simulink model "W07_wpt_los"  (R2024b)
settings: Solver=ode4  StartTime=0  StopTime=T_wpt  FixedStep=h  RelTol=1e-3
InitFcn:
  | addpath(fullfile(fileparts(fileparts(fileparts(get_param(bdroot, 'FileName')))), '_tools'), fileparts(get_param(bdroot, 'FileName'))); run_alone('W07', bdroot);
StopFcn:
  | W07_plot_wpt;
values from neighbouring files (symbols this model uses):
  alpha_lim = cfg.alpha_max(1)    [W07_0_setup.m]
  animate = 1    [W07_0_setup.m]    (also in W07_alloc_run.m = 0; W07_pose_run.m = 0; W07_wpt_run.m = 0)
  B_alloc = cfg.B    [W07_0_setup.m]
  beta_c = pi/2    (= 1.57079632679)    [W07_0_setup.m]
  Delta = 5    [W07_0_setup.m]
  eps_reg = 1e-4    (= 0.0001)    [W07_0_setup.m]    (also in W07_alloc_run.m)
  h = 0.02    [W07_0_setup.m]    (also in W07_3_build_wpt.m = add_line(sys, [a; via; b]); W07_4_build_pose.m = add_line(sys, [a; via; b]))
  k_neg = cfg.k_neg    [W07_0_setup.m]
  k_pos = cfg.k_pos    [W07_0_setup.m]
  Kb = 1    [W07_0_setup.m]
  Kd = 100    [W07_0_setup.m]
  Ki_u = 200    [W07_0_setup.m]
  Kp = 300    [W07_0_setup.m]
  Kp_u = 200    [W07_0_setup.m]
  mp = 25    [W07_0_setup.m]
  N_lim = 150    [W07_0_setup.m]
  n_max = cfg.n_max    [W07_0_setup.m]    (also in W07_plot_ca.m = base_num('n_max',      103.93); W07_plot_sat.m = base_var('n_max',      103.931))
  n_min = cfg.n_min    [W07_0_setup.m]    (also in W07_plot_ca.m = base_num('n_min',     -101.74); W07_plot_sat.m = base_var('n_min',     -101.737))
  Q_tau = eye(3)    [W07_0_setup.m]    (also in W07_alloc_run.m)
  quad = [cfg.pos ; cfg.alpha_max ; cfg.mount]    [W07_0_setup.m]
  R_switch = 3    [W07_0_setup.m]
  rp = [0.05 0 -0.35]'    [W07_0_setup.m]
  stop_at_end = 1    [W07_0_setup.m]
  stop_hold = 15    [W07_0_setup.m]
  T_neg = cfg.k_neg * cfg.n_min^2    [W07_0_setup.m]    (also in W07_plot_ca.m = base_num('T_neg',       66.708); W07_plot_sat.m = base_var('T_neg',        66.708))
  T_pos = cfg.k_pos * cfg.n_max^2    [W07_0_setup.m]    (also in W07_plot_ca.m = base_num('T_pos',      119.682); W07_plot_sat.m = base_var('T_pos',       119.682))
  u_d = 1.0    (= 1)    [W07_0_setup.m]    (also in W07_plot_pose.m = y(:,10))
  V_c = 0.0    (= 0)    [W07_0_setup.m]
  W_alloc = diag(repmat([1 10], 1, 4))    [W07_0_setup.m]
  WP_E = [0   0  60  60  120]'    [W07_0_setup.m]    (also in W07_plot_wpt.m = base_var('WP_E', [0;0;60;60;120]))
  WP_N = [0  60  60   0   60]'    [W07_0_setup.m]    (also in W07_plot_wpt.m = base_var('WP_N', [0;60;60;0;60]))
  x0 = zeros(12,1)    [W07_0_setup.m]
  X_max = 120    [W07_0_setup.m]
settings Model: Creator=admin  LastModifiedBy=admin
settings DataIOCC: ReturnWorkspaceOutputs=off

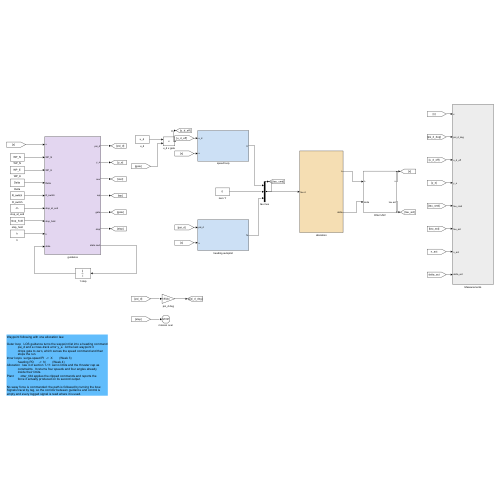
[thumbnail: Simulink's stored preview of the top-level diagram]
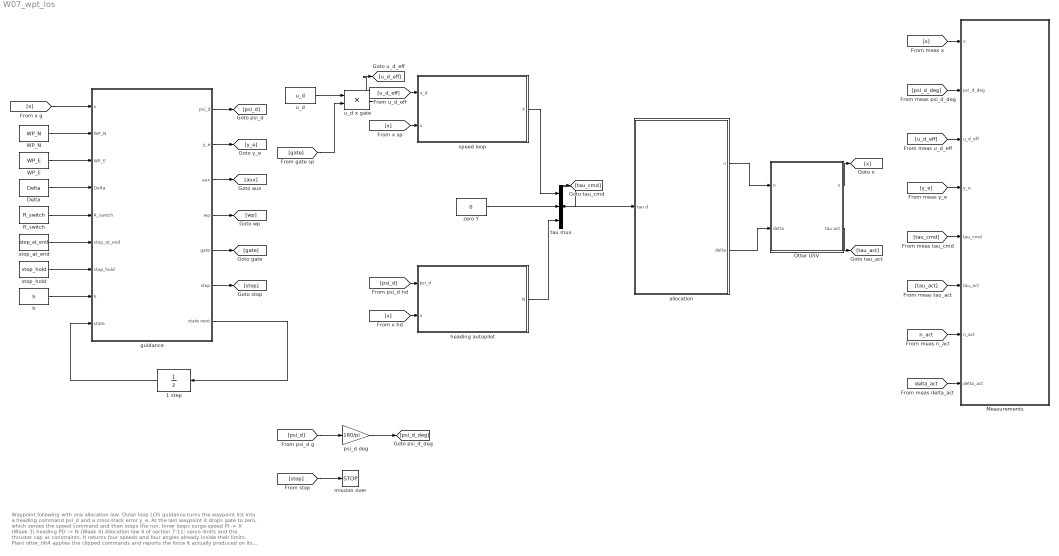
== system W07_wpt_los ==
  note: Waypoint following with one allocation law.
      |
      | Outer loop   LOS guidance turns the waypoint list into a heading command
      |              psi_d and a cross-track error y_e.  At the last waypoint it
      |              drops gate to zero, which zeroes the speed command and then
      |              stops the run.
      | Inner loops  surge-speed PI  ->  X        (Week 3)
      |              heading PD      ->  N        (Week 4)
      | Allocation   law 4 of section 7-11: servo limits and the thruster cap as
      |              constraints.  It returns four speeds and four angles already
      |              inside their limits.
      | Plant        otter_tilt4 applies the clipped commands and reports the
      |              force it actually produced on its second output.
      |
      | No sway force is commanded: the path is followed by turning the bow.
      | Signals travel by tag, so the corridor between guidance and control is
      | empty and every logged signal is read where it is used.
  1 step : UnitDelay  InitialCondition=[1;0]  SampleTime=h  HasFrameUpgradeWarning=on
  Delta : Constant  Value=Delta
  Measurements : Subsystem
  Otter USV : Subsystem
  R_switch : Constant  Value=R_switch
  WP_E : Constant  Value=WP_E
  WP_N : Constant  Value=WP_N
  allocation : Subsystem
  guidance : Subsystem
  h : Constant  Value=h
  heading autopilot : Subsystem
  mission over : Stop
  psi_d deg : Gain  Gain=180/pi
  speed loop : Subsystem
  stop_at_end : Constant  Value=stop_at_end
  stop_hold : Constant  Value=stop_hold
  tau mux : Mux  Inputs=3
  u_d : Constant  Value=u_d
  u_d x gate : Product
  zero Y : Constant  Value=0
  wires:
  [x] -> guidance/1(x)
  WP_N/1 -> guidance/2(WP_N)
  WP_E/1 -> guidance/3(WP_E)
  Delta/1 -> guidance/4(Delta)
  R_switch/1 -> guidance/5(R_switch)
  stop_at_end/1 -> guidance/6(stop_at_end)
  stop_hold/1 -> guidance/7(stop_hold)
  h/1 -> guidance/8(h)
  guidance/7(state next) -> 1 step/1
  1 step/1 -> guidance/9(state)
  guidance/1(psi_d) -> [psi_d]
  guidance/2(y_e) -> [y_e]
  guidance/3(aux) -> [aux]
  guidance/4(wp) -> [wp]
  guidance/5(gate) -> [gate]
  guidance/6(stop) -> [stop]
  [psi_d] -> psi_d deg/1
  psi_d deg/1 -> [psi_d_deg]
  u_d/1 -> u_d x gate/1
  [gate] -> u_d x gate/2
  u_d x gate/1 -> [u_d_eff]
  [u_d_eff] -> speed loop/1(u_d)
  [x] -> speed loop/2(x)
  [psi_d] -> heading autopilot/1(psi_d)
  [x] -> heading autopilot/2(x)
  speed loop/1(X) -> tau mux/1
  zero Y/1 -> tau mux/2
  heading autopilot/1(N) -> tau mux/3
  tau mux/1 -> [tau_cmd], allocation/1(tau d)
  allocation/1(n) -> Otter USV/1(n)
  allocation/2(delta) -> Otter USV/2(delta)
  Otter USV/1(x) -> [x]
  Otter USV/2(tau act) -> [tau_act]
  [stop] -> mission over/1
  [x] -> Measurements/1(x)
  [psi_d_deg] -> Measurements/2(psi_d_deg)
  [u_d_eff] -> Measurements/3(u_d_eff)
  [y_e] -> Measurements/4(y_e)
  [tau_cmd] -> Measurements/5(tau_cmd)
  [tau_act] -> Measurements/6(tau_act)
  [n_act] -> Measurements/7(n_act)
  [delta_act] -> Measurements/8(delta_act)

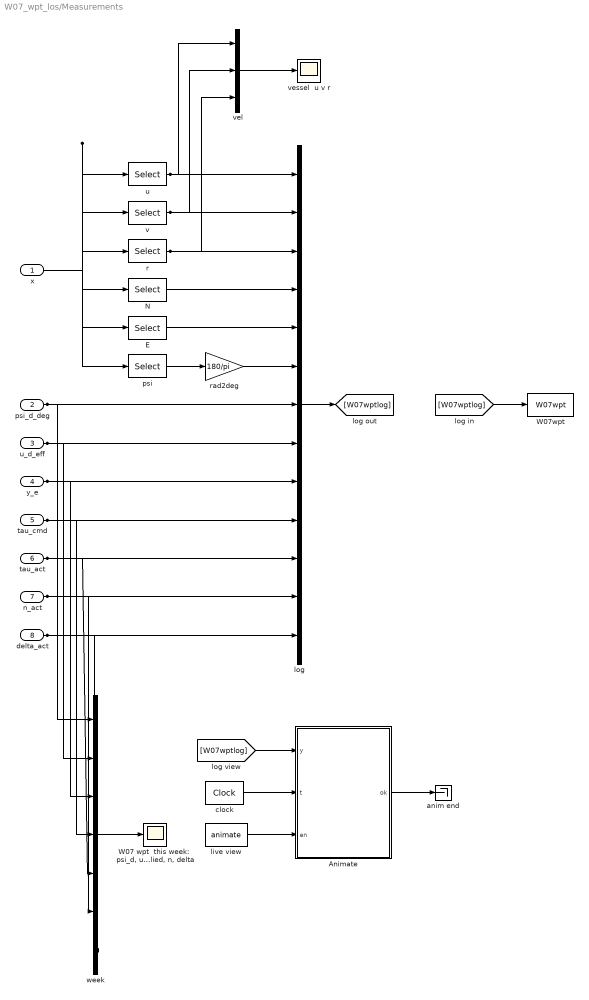
== system W07_wpt_los/Measurements ==
  x : Inport
  psi_d_deg : Inport  Port=2
  u_d_eff : Inport  Port=3
  y_e : Inport  Port=4
  tau_cmd : Inport  Port=5
  tau_act : Inport  Port=6
  n_act : Inport  Port=7
  delta_act : Inport  Port=8
  Animate : MATLAB Function  TreatAsAtomicUnit=on
  E : Selector  InputPortWidth=12  IndexOptions=Index vector (dialog)  Indices=8  OutputSizes=1
  N : Selector  InputPortWidth=12  IndexOptions=Index vector (dialog)  Indices=7  OutputSizes=1
  "W07 wpt  this week:  psi_d, u_d gated, y_e, tau asked and applied, n, delta" : Scope
  W07wpt : ToWorkspace  VariableName=W07wpt  SaveFormat=Structure With Time  SampleTime=-1
  anim end : Terminator
  clock : DigitalClock  SampleTime=h
  live view : Constant  Value=animate
  log : Mux  Inputs=13
  psi : Selector  InputPortWidth=12  IndexOptions=Index vector (dialog)  Indices=12  OutputSizes=1
  r : Selector  InputPortWidth=12  IndexOptions=Index vector (dialog)  Indices=6  OutputSizes=1
  rad2deg : Gain  Gain=180/pi
  u : Selector  InputPortWidth=12  IndexOptions=Index vector (dialog)  Indices=1  OutputSizes=1
  v : Selector  InputPortWidth=12  IndexOptions=Index vector (dialog)  Indices=2  OutputSizes=1
  vel : Mux  Inputs=3
  vessel  u v r : Scope
  week : Mux  Inputs=7
  wires:
  x/1 -> u/1, v/1, r/1, N/1, E/1, psi/1
  log/1 -> [W07wptlog]
  [W07wptlog] -> W07wpt/1
  psi/1 -> rad2deg/1
  u/1 -> log/1, vel/1
  v/1 -> log/2, vel/2
  r/1 -> log/3, vel/3
  N/1 -> log/4
  E/1 -> log/5
  rad2deg/1 -> log/6
  psi_d_deg/1 -> log/7, week/1
  u_d_eff/1 -> log/8, week/2
  y_e/1 -> log/9, week/3
  tau_cmd/1 -> log/10, week/4
  tau_act/1 -> log/11, week/5
  n_act/1 -> log/12, week/6
  delta_act/1 -> log/13, week/7
  vel/1 -> vessel  u v r/1
  week/1 -> "W07 wpt  this week:  psi_d, u_d gated, y_e, tau asked and applied, n, delta"/1
  [W07wptlog] -> Animate/1(y)
  clock/1 -> Animate/2(t)
  live view/1 -> Animate/3(en)
  Animate/1(ok) -> anim end/1

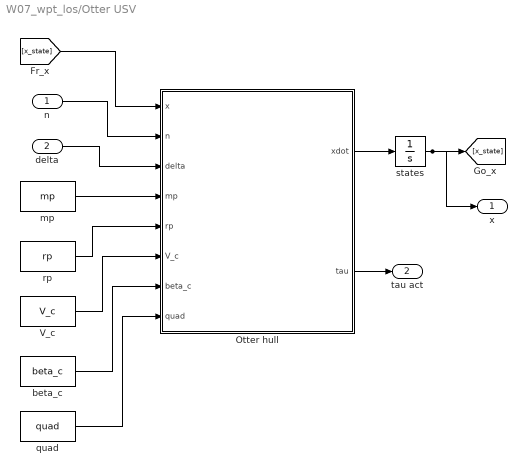
== system W07_wpt_los/Otter USV ==
  n : Inport
  delta : Inport  Port=2
  Otter hull : MATLAB Function  TreatAsAtomicUnit=on
  V_c : Constant  Value=V_c
  beta_c : Constant  Value=beta_c
  mp : Constant  Value=mp
  quad : Constant  Value=quad
  rp : Constant  Value=rp
  states : Integrator  InitialCondition=x0
  x : Outport
  tau act : Outport  Port=2
  wires:
  [x_state] -> Otter hull/1(x)
  mp/1 -> Otter hull/4(mp)
  quad/1 -> Otter hull/8(quad)
  beta_c/1 -> Otter hull/7(beta_c)
  n/1 -> Otter hull/2(n)
  V_c/1 -> Otter hull/6(V_c)
  delta/1 -> Otter hull/3(delta)
  rp/1 -> Otter hull/5(rp)
  Otter hull/1(xdot) -> states/1
  Otter hull/2(tau) -> tau act/1
  states/1 -> x/1, [x_state]

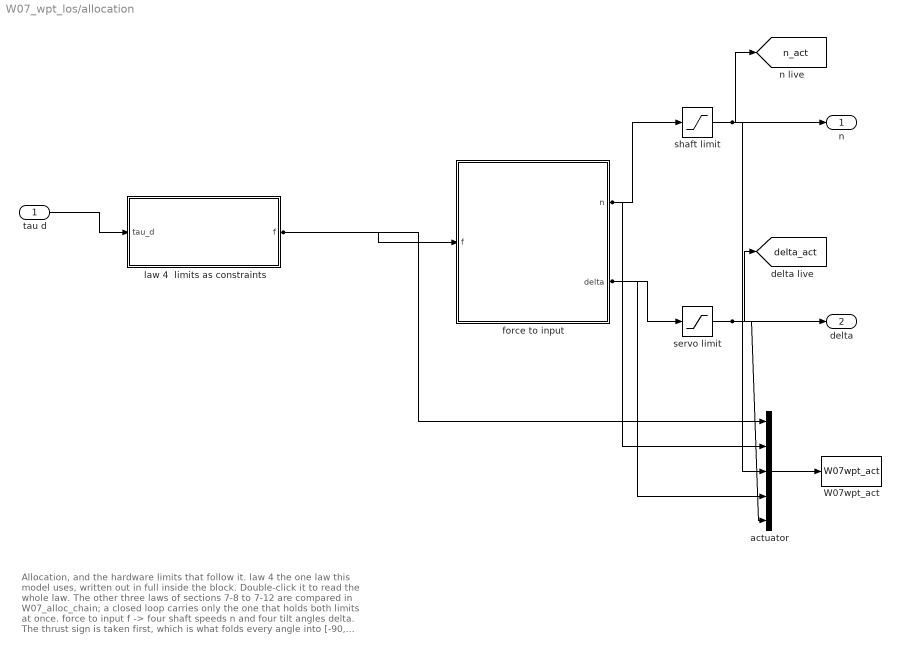
== system W07_wpt_los/allocation ==
  note: Allocation, and the hardware limits that follow it.
      |
      | law 4             the one law this model uses, written out in full
      |                   inside the block. Double-click it to read the whole law.
      |                   The other three laws of sections 7-8 to 7-12 are compared
      |                   in W07_alloc_chain; a closed loop carries only the one
      |                   that holds both limits at once.
      | force to input    f -> four shaft speeds n and four tilt angles delta. The
      |                   thrust sign is taken first, which is what folds every
      |                   angle into [-90, +90] deg before the servo ever sees it.
      |                   A unit asked for less than 0.5 N is held at n = 0 and
      |                   delta = 0, because below that the angle is arithmetic
      |                   noise and the servo would chatter at rest.
      | shaft limit       n clipped to [n_min, n_max].
      | servo limit       delta clipped to +-alpha_lim.
      | n live            the two clipped commands also leave as the global tags
      | delta live        n_act and delta_act, so the live view can draw them
      |                   against their limits while the run is still going. The
      |                   record below is readable only after it ends.
      | actuator          the record of this solve, written to W07wpt_act as 24
      |                   columns:  f(8),  n asked(4),  n allowed(4),  delta
      |                   asked(4),  delta allowed(4). Wherever asked and allowed
      |                   differ, that unit is against a limit.
      |
      | What the hull was actually given is not rebuilt here: the motion model
      | already forms it from the clipped n and delta and reports it on its own
      | second output.
  tau d : Inport
  W07wpt_act : ToWorkspace  VariableName=W07wpt_act  SampleTime=-1
  actuator : Mux  Inputs=5
  force to input : MATLAB Function  TreatAsAtomicUnit=on
  law 4  limits as constraints : MATLAB Function  TreatAsAtomicUnit=on
  servo limit : Saturate  UpperLimit=alpha_lim  LowerLimit=-alpha_lim
  shaft limit : Saturate  UpperLimit=n_max  LowerLimit=n_min
  n : Outport
  delta : Outport  Port=2
  tag scope: delta_act=global, n_act=global
  wires:
  tau d/1 -> law 4  limits as constraints/1(tau_d)
  law 4  limits as constraints/1(f) -> force to input/1(f), actuator/1
  force to input/1(n) -> shaft limit/1, actuator/2
  force to input/2(delta) -> servo limit/1, actuator/4
  shaft limit/1 -> n/1, [n_act], actuator/3
  servo limit/1 -> delta/1, [delta_act], actuator/5
  actuator/1 -> W07wpt_act/1

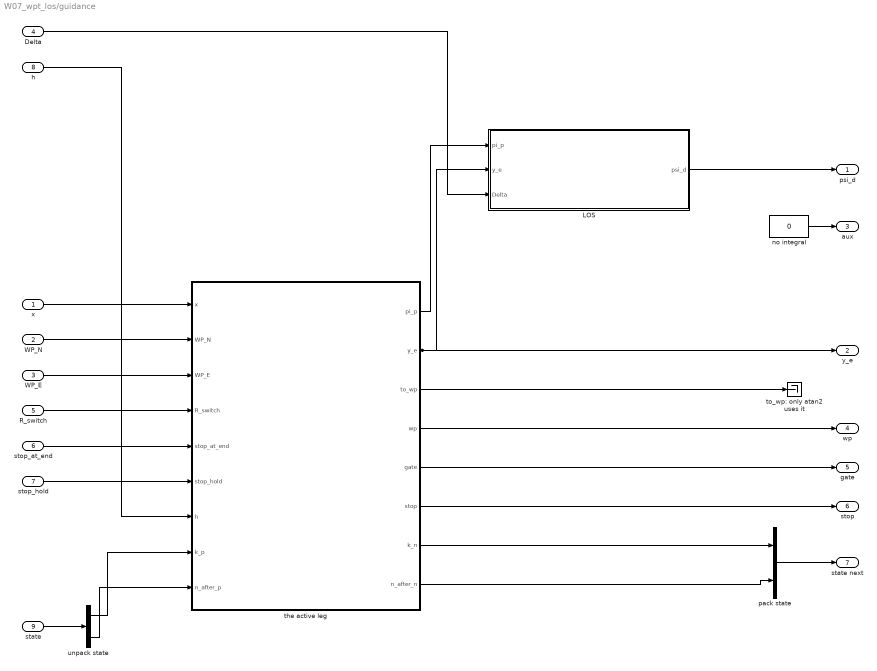
== system W07_wpt_los/guidance ==
  x : Inport
  WP_N : Inport  Port=2
  WP_E : Inport  Port=3
  Delta : Inport  Port=4
  R_switch : Inport  Port=5
  stop_at_end : Inport  Port=6
  stop_hold : Inport  Port=7
  h : Inport  Port=8
  state : Inport  Port=9
  LOS : MATLAB Function  TreatAsAtomicUnit=on
  no integral : Constant  Value=0
  pack state : Mux  Inputs=2
  the active leg : MATLAB Function  TreatAsAtomicUnit=on
  to_wp: only atan2 uses it : Terminator
  unpack state : Demux  Outputs=2
  psi_d : Outport
  y_e : Outport  Port=2
  aux : Outport  Port=3
  wp : Outport  Port=4
  gate : Outport  Port=5
  stop : Outport  Port=6
  state next : Outport  Port=7
  wires:
  x/1 -> the active leg/1(x)
  WP_N/1 -> the active leg/2(WP_N)
  WP_E/1 -> the active leg/3(WP_E)
  R_switch/1 -> the active leg/4(R_switch)
  stop_at_end/1 -> the active leg/5(stop_at_end)
  stop_hold/1 -> the active leg/6(stop_hold)
  h/1 -> the active leg/7(h)
  state/1 -> unpack state/1
  unpack state/1 -> the active leg/8(k_p)
  unpack state/2 -> the active leg/9(n_after_p)
  the active leg/1(pi_p) -> LOS/1(pi_p)
  the active leg/2(y_e) -> LOS/2(y_e), y_e/1
  Delta/1 -> LOS/3(Delta)
  the active leg/3(to_wp) -> to_wp: only atan2 uses it/1
  the active leg/7(k_n) -> pack state/1
  the active leg/8(n_after_n) -> pack state/2
  LOS/1(psi_d) -> psi_d/1
  no integral/1 -> aux/1
  the active leg/4(wp) -> wp/1
  the active leg/5(gate) -> gate/1
  the active leg/6(stop) -> stop/1
  pack state/1 -> state next/1

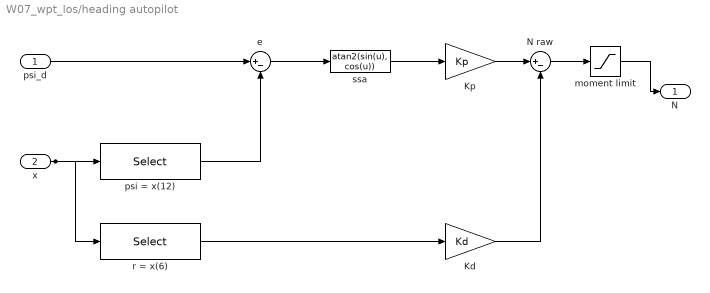
== system W07_wpt_los/heading autopilot ==
  psi_d : Inport
  x : Inport  Port=2
  Kd : Gain  Gain=Kd
  Kp : Gain  Gain=Kp
  N raw : Sum  Inputs=|+-
  e : Sum  Inputs=|+-
  moment limit : Saturate  UpperLimit=N_lim  LowerLimit=-N_lim
  psi = x(12) : Selector  InputPortWidth=12  IndexOptions=Index vector (dialog)  Indices=12  OutputSizes=1
  r = x(6) : Selector  InputPortWidth=12  IndexOptions=Index vector (dialog)  Indices=6  OutputSizes=1
  ssa : Fcn  Expr=atan2(sin(u), cos(u))
  N : Outport
  wires:
  x/1 -> psi = x(12)/1, r = x(6)/1
  psi_d/1 -> e/1
  psi = x(12)/1 -> e/2
  e/1 -> ssa/1
  ssa/1 -> Kp/1
  r = x(6)/1 -> Kd/1
  Kp/1 -> N raw/1
  Kd/1 -> N raw/2
  N raw/1 -> moment limit/1
  moment limit/1 -> N/1

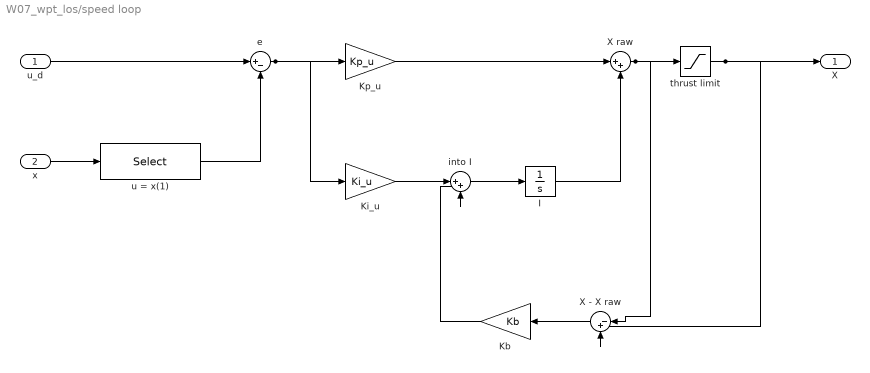
== system W07_wpt_los/speed loop ==
  u_d : Inport
  x : Inport  Port=2
  I : Integrator
  Kb : Gain  Gain=Kb
  Ki_u : Gain  Gain=Ki_u
  Kp_u : Gain  Gain=Kp_u
  X - X raw : Sum  Inputs=|-+
  X raw : Sum  Inputs=|++
  e : Sum  Inputs=|+-
  into I : Sum  Inputs=|++
  thrust limit : Saturate  UpperLimit=X_max  LowerLimit=-X_max
  u = x(1) : Selector  InputPortWidth=12  IndexOptions=Index vector (dialog)  Indices=1  OutputSizes=1
  X : Outport
  wires:
  x/1 -> u = x(1)/1
  u_d/1 -> e/1
  u = x(1)/1 -> e/2
  e/1 -> Kp_u/1, Ki_u/1
  Ki_u/1 -> into I/1
  into I/1 -> I/1
  Kp_u/1 -> X raw/1
  I/1 -> X raw/2
  X raw/1 -> thrust limit/1, X - X raw/1
  thrust limit/1 -> X/1, X - X raw/2
  X - X raw/1 -> Kb/1
  Kb/1 -> into I/2

== matlab function W07_wpt_los/guidance/the active leg ==
  settings: updateMethod=DISCRETE  sampleTime=h
  data: x input; pi_p output double size=[1 1]; WP_N input; WP_E input; R_switch input; stop_at_end input; stop_hold input; h input; k_p input; n_after_p input; y_e output; to_wp output; wp output; gate output; stop output; k_n output; n_after_n output
function [pi_p, y_e, to_wp, wp, gate, stop, k_n, n_after_n] = active_leg(x, WP_N, WP_E, R_switch, stop_at_end, stop_hold, h, k_p, n_after_p)
%#codegen
%ACTIVE_LEG  어느 다리를 따라가는 중인가, 그 다리에서 얼마나 벗어났는가,
%            그리고 다음 다리로 넘어갈 때가 되었는가.
%            Which leg is being followed, how far off it the vessel is, and
%            whether it is time to move to the next leg.
%
%   유도 법칙이 무엇이든 이 계산은 같다. 법칙은 여기서 나온 pi_p 와 y_e 로
%   **겨냥하는 방법**만 정한다.
%   This is the same for every guidance law; a law only decides how to aim,
%   given the pi_p and y_e computed here.
%
%   입력 x 는 Otter 의 12 상태 (위치 N = x(7), E = x(8)).
%   The input x is the Otter 12 states, with position N = x(7), E = x(8).
%
%   출력 / outputs
%     pi_p       지금 다리의 방향 [rad] / the direction of the active leg
%     y_e        그 다리에서 옆으로 벗어난 거리 [m], 오른쪽이 +
%                distance off that leg, to the right positive
%     to_wp      배에서 다음 웨이포인트까지의 벡터 [dN; dE] - 법칙 1 만 쓴다
%                the vector to the next waypoint; only law 1 uses it
%     wp         지금 따라가는 다리 번호 / the leg being followed
%     gate       속도 명령에 곱하는 0/1. 임무가 끝나면 0 이 되어 배가 선다
%                0/1 multiplying the speed command: 0 once the mission is over
%     stop       시뮬레이션을 끝내라는 0/1 / 0/1 asking the run to end

% 0) 기억하는 값 둘이 **포트로 들어온다**: 지금 다리 k, 도착 뒤 스텝 수.
%    둘 다 **직전 스텝의** 값이다 - 캔버스의 Unit Delay 가 들고 있다가 돌려준다.
%    The two remembered values arrive through ports, and both are the values of
%    the PREVIOUS step: the Unit Delay on the canvas held them.
%
%    순서가 persistent 판과 비트 단위로 같게 만든다 / the order makes this exact
%      pi_p, x_e, y_e 와 to_wp 는 **옛** 다리로, wp 와 gate 는 **새** 다리로
%      구한다. 그래서 한 스텝의 모든 출력이 (x, 직전 상태) 만의 함수다.
%      The errors and to_wp come from the OLD leg, wp and the gate from the NEW
%      one, so every output of a step is a function of (x, previous state).
k = round(k_p);
n = numel(WP_N);
%    신호로 들어온 지표를 범위 안에 가둔다. 실제로 도달하는 값 위에서는 항등이다.
%    Clamp the index that arrives as a signal; the identity map on every value
%    it can actually take.
if k < 1, k = 1; end
if k > n-1, k = n-1; end
n_after = n_after_p;
N = x(7);  E = x(8);

% 1) 지금 다리: 웨이포인트 k 에서 k+1 로. 그 방향이 경로 각 pi_p 다.
%    The active leg runs from waypoint k to k+1; its direction is pi_p.
kn = min(k+1, n);
Nk = WP_N(k);   Ek = WP_E(k);
Nn = WP_N(kn);  En = WP_E(kn);
pi_p = atan2(En - Ek, Nn - Nk);

% 2) 배의 위치를 경로 좌표로 돌린다: x_e = 다리를 따라 간 거리,
%    y_e = 다리에서 옆으로 벗어난 거리.
%    Rotate the position into path coordinates: x_e along the leg, y_e off it.
dN = N - Nk;  dE = E - Ek;
x_e =  dN*cos(pi_p) + dE*sin(pi_p);
y_e = -dN*sin(pi_p) + dE*cos(pi_p);

%    법칙 1 이 쓰는 벡터. 선이 아니라 점을 겨냥하는 법칙이라 이것만 필요하다.
%    The vector law 1 uses: it aims at a point, not at the line, so this is all
%    it needs.
to_wp = [Nn - N; En - E];

% 3) 다리 끝까지 R_switch 보다 적게 남으면 다음 다리로 (MSS 와 같은 판정).
%    With less than R_switch left to the end of the leg, move on (as MSS does).
d = sqrt((Nn - Nk)^2 + (En - Ek)^2);
near_end = (d - x_e) < R_switch;
if near_end && k < n-1
    k = k + 1;
    near_end = false;          % 새 다리는 방금 시작했다 / the new leg has just begun
end
wp = k;

% 4) 임무의 끝. **마지막 다리**에서 같은 판정이 참이 되면 더 갈 곳이 없다.
%    다음 다리로 넘어가는 대신 속도 명령을 0 으로 내리고, stop_hold 초 뒤에
%    실행을 끝낸다. 그 몇 초는 배가 서는 모습을 보기 위한 것이다.
%    stop_at_end = 0 이면 둘 다 하지 않는다.
%    The end of the mission: when the same test becomes true on the LAST leg
%    there is nowhere to switch to, so the speed command is taken to zero and
%    the run ends stop_hold seconds later - seconds that are there so the
%    vessel can be seen slowing down. With stop_at_end = 0 neither happens.
arrived = near_end && k == n-1;
if arrived
    n_after = n_after + 1;
end
gate = 1;
stop = 0;
if stop_at_end > 0.5
    if n_after > 0
        gate = 0;
    end
    if n_after * h > stop_hold
        stop = 1;
    end
end

% 5) 다음 스텝으로 넘길 상태 / the state handed to the Unit Delay
k_n       = k;
n_after_n = n_after;
end

== matlab function W07_wpt_los/guidance/LOS ==
  settings: updateMethod=DISCRETE  sampleTime=h
  data: pi_p input; psi_d output double size=[1 1]; y_e input; Delta input
function psi_d = los(pi_p, y_e, Delta)
%#codegen
%LOS  법칙 2 — 경로 위에서 Delta 만큼 앞의 점을 겨냥한다.
%     Law 2: aim at the point Delta ahead on the path.
%
%         psi_d = pi_p - atan(y_e / Delta)
%
%   두 항이 각각 할 일이 있다. pi_p 는 "경로와 나란히 서라", atan 은 "벗어난
%   만큼 경로 쪽으로 기울여라".
%   The two terms each have a job: pi_p says "line up with the path", the atan
%   says "lean towards it by how far off you are".
%
%   y_e 가 작으면 atan(y_e/Delta) ~ y_e/Delta 이므로, 이것은 횡방향 오차에
%   대한 **P 제어기**이고 이득은 Kp = 1/Delta 다. Delta 를 줄이면 이득이
%   커진다 - P 제어기와 똑같이 빨라지다가 떨린다.
%   For small y_e, atan(y_e/Delta) ~ y_e/Delta: a P controller on the
%   cross-track error with Kp = 1/Delta. A smaller Delta is a larger gain, and
%   behaves like one - quicker, then oscillatory.
psi_d = pi_p - atan(y_e / Delta);
end

== matlab function W07_wpt_los/allocation/law 4  limits as constraints ==
  data: tau_d input; f output double size=[8 1]; B_alloc parameter; W_alloc parameter; alpha_lim parameter; Q_tau parameter; eps_reg parameter; T_pos parameter; T_neg parameter
function f = law4_limits_as_constraints(tau_d, B_alloc, W_alloc, alpha_lim, Q_tau, eps_reg, T_pos, T_neg)
% LAW 4 -- the servo limit AND the thrust cap as hard constraints.  7-12.
%
% Minimise   ||Q (B f - tau_d)||^2 + eps ||W^(1/2) f||^2
% subject to, for every unit i,
%
%     |f_yi| <= tan(alpha_lim) sigma_i f_xi               the servo limit
%     cos(th) x' + sin(th) y' <= R cos(alpha_lim/M)       the thrust cap
%
% written in unit axes x' = sigma_i f_xi and y' = sigma_i f_yi. Both are
% straight lines once the thrust sign sigma_i of that unit is fixed, so the
% problem is a QP: no local minima. The signs are not known in advance, so
% all 2^4 = 16 sign combinations are solved and the cheapest feasible one is
% kept. tau_d sits in the cost rather than in an equality, so a solution
% exists even when the demand cannot be delivered.
%
% The cap is an arc, which no QP can hold. It is replaced by M = 3 inscribed
% chords: neighbouring chords meet exactly on the circle of radius R and
% their midpoints sit at cos(15 deg) = 0.966 R, so the polygon never breaks
% the cap and is at worst 3.4 per cent conservative.
%
% lsqlin has no code generation support, so the call is extrinsic and every
% output it returns is given a size and a type beforehand.
coder.extrinsic('lsqlin', 'optimoptions');

M = 3;                   % chords per cone, the n_chord of W07_vars
t = tan(alpha_lim);

% the whole cost as one least-squares residual,  ||C f - d||
C = [Q_tau*B_alloc ; sqrt(eps_reg)*sqrt(W_alloc)];
d = [Q_tau*tau_d   ; zeros(8,1)];

% the fallback, used if no sign combination turns out to be feasible
Wi = W_alloc \ eye(8);
f  = Wi * B_alloc' * ((B_alloc*Wi*B_alloc') \ tau_d);

opts = optimoptions('lsqlin', 'Display', 'off');
best = inf;

for p = 0:15
    % the four thrust signs of combination p, read off its four bits
    sg = zeros(4,1);
    for i = 1:4
        sg(i) = 1 - 2*mod(floor(p/2^(i-1)), 2);
    end

    A = zeros(4*(2+M), 8);
    b = zeros(4*(2+M), 1);
    r = 0;
    for i = 1:4
        s = sg(i);
        if s > 0
            R = T_pos;
        else
            R = T_neg;    % written positive, so the cap is a radius
        end
        r = r + 1;  A(r, 2*i-1) = -t*s;  A(r, 2*i) =  1;
        r = r + 1;  A(r, 2*i-1) = -t*s;  A(r, 2*i) = -1;
        for j = 1:M
            th = -alpha_lim + (j - 0.5)*(2*alpha_lim/M);
            r  = r + 1;
            A(r, 2*i-1) = s*cos(th);
            A(r, 2*i)   = s*sin(th);
            b(r)        = R*cos(alpha_lim/M);
        end
    end

    x   = zeros(8,1);
    cst = 0;
    res = zeros(11,1);
    ef  = 0;
    [x, cst, res, ef] = lsqlin(C, d, A, b, [], [], [], [], [], opts);

    % a cost is a cost only where the solver reported a solution
    if ef > 0 && cst < best
        best = cst;
        f    = x;
    end
end
end

== matlab function W07_wpt_los/allocation/force to input ==
  data: f input; n output double size=[4 1]; delta output; k_pos parameter; k_neg parameter
function [n, delta] = force2input(f, k_pos, k_neg)
% Eight force components -> four shaft speeds and four tilt angles.
%
%     sigma_i = sign(f_xi)                        which way the unit pushes
%     T_i     = sigma_i |f_i|                     signed thrust        [N]
%     delta_i = atan2(sigma_i f_yi, sigma_i f_xi) tilt angle         [rad]
%     n_i     = sign(T_i) sqrt(|T_i| / k_i)       shaft speed      [rad/s]
%
% Multiplying BOTH arguments of atan2 by sigma_i turns the direction through
% exactly pi, and because sigma_i f_xi >= 0 the result always lands in
% [-pi/2, +pi/2]. That is what keeps the angle reachable: a unit pushing
% astern comes out as negative thrust at a small angle instead of positive
% thrust at 180 deg, which no servo limited to +-45 deg could hold.
fx = f(1:2:7);
fy = f(2:2:8);
s  = sign(fx);
s(s == 0) = 1;      % a unit with no surge component is left pointing abeam

T     = s .* hypot(fx, fy);
delta = atan2(s.*fy, s.*fx);

% The coefficient depends on the sign because a propeller pushing astern is
% less efficient than the same propeller pushing ahead.
k = k_pos*double(T >= 0) + k_neg*double(T < 0);
n = sign(T) .* sqrt(abs(T) ./ k);

% Below a tiny force the angle stops meaning anything: atan2 of two numbers
% near zero turns with the last bit of the arithmetic, so a servo asked to
% follow it would chatter while the vessel sits still. Hold such a unit at
% zero instead. The threshold is 0.5 N, which is 0.4 % of the ahead cap, so
% no force a controller could usefully ask for is thrown away here.
tiny = hypot(fx, fy) < 0.5;
delta(tiny) = 0;
n(tiny)     = 0;
end

== matlab function W07_wpt_los/Otter USV/Otter hull ==
  data: x input; xdot output double size=[12 1]; n input; delta input; mp input; rp input; V_c input; beta_c input; quad input; tau output double size=[3 1]
function [xdot, tau] = otter_hull(x, n, delta, mp, rp, V_c, beta_c, quad)
% otter_tilt4.m: Fossen's otter.m with four tilting thrusters, called
% unchanged from _tools. Four shaft speeds and four angles in, tau built
% inside, in the same four marked places as otter_bow.m.
%
%   x      12 states, fed back from the integrator
%   n      shaft speeds [rad/s], fore port / fore stbd / aft port / aft stbd
%   delta  tilt angles [rad], measured from the body x axis, CCW positive
%   quad   3 x 4: the x stations, the y stations and the tilt limits
%
% Rows 1, 2 and 6 of tau all carry the angles, by the column rule
% [e_x; e_y; x e_y - y e_x] with e = [cos delta; sin delta]. Nothing is
% added after the call; there is no superposition and no tau_ext port.
%
% The second output is the [X; Y; N] the model actually used, formed after n
% and delta are clipped to their limits. It is the delivered force, so no
% block outside has to rebuild it from n and delta.
%
% otter_tilt4.m is not written for code generation, so the call is extrinsic
% and both outputs have to be pre-sized for Simulink to know their widths.
coder.extrinsic('otter_tilt4');

xdot = zeros(12,1);
spd  = 0;
tau  = zeros(3,1);
[xdot, spd, tau] = otter_tilt4(x, n, delta, mp, rp, V_c, beta_c, quad);
end

== matlab function W07_wpt_los/Measurements/Animate ==
  data: y input; ok output; t input; en input
function ok = Animate(y, t, en)
%#codegen
% Live view of the vessel while the model runs.
%
% A MATLAB Function block cannot plot, so the drawing function is declared
% extrinsic: Simulink calls plain MATLAB rather than generating code for it.
% Set animate = 0 in the setup script to switch the live view off.
%
% y is the whole log vector, in the column order this subsystem builds:
% [u v r N E psi] first, psi in DEGREES, then the week's own signals.
% The wrapper names the columns; nothing else counts them.
coder.extrinsic('W07wpt_animate');
ok = 1;
if en > 0.5
    W07wpt_animate(y, t);
end
end
